simulink model "rfsoc4x2_ospfb_128"  (R2021a)
settings: Solver=VariableStepAuto  StartTime=0.0  StopTime=2048  RelTol=1e-3
undefined symbols (not defined in the file): pfb_coeff_gen_calc
libraries: xbsIndex_r4 x37092, casper_library_delays x737, casper_library_misc x68, xps_library x1
(part 83 of 339)

== system rfsoc4x2_ospfb_128/pfb_fir_real6/adder_1_12 ==
  sync : Inport
  din1 : Inport  Port=2
  din2 : Inport  Port=3
  din3 : Inport  Port=4
  din4 : Inport  Port=5
  addr1 : xbsIndex_r4/AddSub  mode=Addition  use_carryin=off  use_carryout=off  en=off  latency=1  precision=User Defined  arith_type="Signed  (2's comp)"  n_bits=32  bin_pt=30  quantization=Truncate  overflow=Wrap  use_behavioral_HDL=on  hw_selection=Fabric  pipelined=on  use_rpm=on  dbl_ovrd=off  block_type=addsub
  addr2 : xbsIndex_r4/AddSub  mode=Addition  use_carryin=off  use_carryout=off  en=off  latency=1  precision=User Defined  arith_type="Signed  (2's comp)"  n_bits=32  bin_pt=30  quantization=Truncate  overflow=Wrap  use_behavioral_HDL=on  hw_selection=Fabric  pipelined=on  use_rpm=on  dbl_ovrd=off  block_type=addsub
  addr3 : xbsIndex_r4/AddSub  mode=Addition  use_carryin=off  use_carryout=off  en=off  latency=1  precision=User Defined  arith_type="Signed  (2's comp)"  n_bits=32  bin_pt=30  quantization=Truncate  overflow=Wrap  use_behavioral_HDL=off  hw_selection=Fabric  pipelined=on  use_rpm=on  dbl_ovrd=off  block_type=addsub
  sync_delay : xbsIndex_r4/Delay  rst=off  infoeditControl=Selection of Reset will increase slice count due to use of real FFs and instead of SRLs  en=off  latency=2  reg_retiming=on  dbl_ovrd=off  block_type=delay
      settings: block_version=11.4
  sync_out : Outport  VectorParamsAs1DForOutWhenUnconnected=off
  dout : Outport  Port=2  VectorParamsAs1DForOutWhenUnconnected=off
  wires:
  sync/1 -> sync_delay/1
  sync_delay/1 -> sync_out/1
  din1/1 -> addr1/1
  din2/1 -> addr1/2
  din3/1 -> addr2/1
  din4/1 -> addr2/2
  addr1/1 -> addr3/1
  addr2/1 -> addr3/2
  addr3/1 -> dout/1

== system rfsoc4x2_ospfb_128/pfb_fir_real6/adder_1_13 ==
  sync : Inport
  din1 : Inport  Port=2
  din2 : Inport  Port=3
  din3 : Inport  Port=4
  din4 : Inport  Port=5
  addr1 : xbsIndex_r4/AddSub  mode=Addition  use_carryin=off  use_carryout=off  en=off  latency=1  precision=User Defined  arith_type="Signed  (2's comp)"  n_bits=32  bin_pt=30  quantization=Truncate  overflow=Wrap  use_behavioral_HDL=on  hw_selection=Fabric  pipelined=on  use_rpm=on  dbl_ovrd=off  block_type=addsub
  addr2 : xbsIndex_r4/AddSub  mode=Addition  use_carryin=off  use_carryout=off  en=off  latency=1  precision=User Defined  arith_type="Signed  (2's comp)"  n_bits=32  bin_pt=30  quantization=Truncate  overflow=Wrap  use_behavioral_HDL=on  hw_selection=Fabric  pipelined=on  use_rpm=on  dbl_ovrd=off  block_type=addsub
  addr3 : xbsIndex_r4/AddSub  mode=Addition  use_carryin=off  use_carryout=off  en=off  latency=1  precision=User Defined  arith_type="Signed  (2's comp)"  n_bits=32  bin_pt=30  quantization=Truncate  overflow=Wrap  use_behavioral_HDL=off  hw_selection=Fabric  pipelined=on  use_rpm=on  dbl_ovrd=off  block_type=addsub
  sync_delay : xbsIndex_r4/Delay  rst=off  infoeditControl=Selection of Reset will increase slice count due to use of real FFs and instead of SRLs  en=off  latency=2  reg_retiming=on  dbl_ovrd=off  block_type=delay
      settings: block_version=11.4
  sync_out : Outport  VectorParamsAs1DForOutWhenUnconnected=off
  dout : Outport  Port=2  VectorParamsAs1DForOutWhenUnconnected=off
  wires:
  sync/1 -> sync_delay/1
  sync_delay/1 -> sync_out/1
  din1/1 -> addr1/1
  din2/1 -> addr1/2
  din3/1 -> addr2/1
  din4/1 -> addr2/2
  addr1/1 -> addr3/1
  addr2/1 -> addr3/2
  addr3/1 -> dout/1

== system rfsoc4x2_ospfb_128/pfb_fir_real6/adder_1_14 ==
  sync : Inport
  din1 : Inport  Port=2
  din2 : Inport  Port=3
  din3 : Inport  Port=4
  din4 : Inport  Port=5
  addr1 : xbsIndex_r4/AddSub  mode=Addition  use_carryin=off  use_carryout=off  en=off  latency=1  precision=User Defined  arith_type="Signed  (2's comp)"  n_bits=32  bin_pt=30  quantization=Truncate  overflow=Wrap  use_behavioral_HDL=on  hw_selection=Fabric  pipelined=on  use_rpm=on  dbl_ovrd=off  block_type=addsub
  addr2 : xbsIndex_r4/AddSub  mode=Addition  use_carryin=off  use_carryout=off  en=off  latency=1  precision=User Defined  arith_type="Signed  (2's comp)"  n_bits=32  bin_pt=30  quantization=Truncate  overflow=Wrap  use_behavioral_HDL=on  hw_selection=Fabric  pipelined=on  use_rpm=on  dbl_ovrd=off  block_type=addsub
  addr3 : xbsIndex_r4/AddSub  mode=Addition  use_carryin=off  use_carryout=off  en=off  latency=1  precision=User Defined  arith_type="Signed  (2's comp)"  n_bits=32  bin_pt=30  quantization=Truncate  overflow=Wrap  use_behavioral_HDL=off  hw_selection=Fabric  pipelined=on  use_rpm=on  dbl_ovrd=off  block_type=addsub
  sync_delay : xbsIndex_r4/Delay  rst=off  infoeditControl=Selection of Reset will increase slice count due to use of real FFs and instead of SRLs  en=off  latency=2  reg_retiming=on  dbl_ovrd=off  block_type=delay
      settings: block_version=11.4
  sync_out : Outport  VectorParamsAs1DForOutWhenUnconnected=off
  dout : Outport  Port=2  VectorParamsAs1DForOutWhenUnconnected=off
  wires:
  sync/1 -> sync_delay/1
  sync_delay/1 -> sync_out/1
  din1/1 -> addr1/1
  din2/1 -> addr1/2
  din3/1 -> addr2/1
  din4/1 -> addr2/2
  addr1/1 -> addr3/1
  addr2/1 -> addr3/2
  addr3/1 -> dout/1

== system rfsoc4x2_ospfb_128/pfb_fir_real6/adder_1_15 ==
  sync : Inport
  din1 : Inport  Port=2
  din2 : Inport  Port=3
  din3 : Inport  Port=4
  din4 : Inport  Port=5
  addr1 : xbsIndex_r4/AddSub  mode=Addition  use_carryin=off  use_carryout=off  en=off  latency=1  precision=User Defined  arith_type="Signed  (2's comp)"  n_bits=32  bin_pt=30  quantization=Truncate  overflow=Wrap  use_behavioral_HDL=on  hw_selection=Fabric  pipelined=on  use_rpm=on  dbl_ovrd=off  block_type=addsub
  addr2 : xbsIndex_r4/AddSub  mode=Addition  use_carryin=off  use_carryout=off  en=off  latency=1  precision=User Defined  arith_type="Signed  (2's comp)"  n_bits=32  bin_pt=30  quantization=Truncate  overflow=Wrap  use_behavioral_HDL=on  hw_selection=Fabric  pipelined=on  use_rpm=on  dbl_ovrd=off  block_type=addsub
  addr3 : xbsIndex_r4/AddSub  mode=Addition  use_carryin=off  use_carryout=off  en=off  latency=1  precision=User Defined  arith_type="Signed  (2's comp)"  n_bits=32  bin_pt=30  quantization=Truncate  overflow=Wrap  use_behavioral_HDL=off  hw_selection=Fabric  pipelined=on  use_rpm=on  dbl_ovrd=off  block_type=addsub
  sync_delay : xbsIndex_r4/Delay  rst=off  infoeditControl=Selection of Reset will increase slice count due to use of real FFs and instead of SRLs  en=off  latency=2  reg_retiming=on  dbl_ovrd=off  block_type=delay
      settings: block_version=11.4
  sync_out : Outport  VectorParamsAs1DForOutWhenUnconnected=off
  dout : Outport  Port=2  VectorParamsAs1DForOutWhenUnconnected=off
  wires:
  sync/1 -> sync_delay/1
  sync_delay/1 -> sync_out/1
  din1/1 -> addr1/1
  din2/1 -> addr1/2
  din3/1 -> addr2/1
  din4/1 -> addr2/2
  addr1/1 -> addr3/1
  addr2/1 -> addr3/2
  addr3/1 -> dout/1

== system rfsoc4x2_ospfb_128/pfb_fir_real6/adder_1_16 ==
  sync : Inport
  din1 : Inport  Port=2
  din2 : Inport  Port=3
  din3 : Inport  Port=4
  din4 : Inport  Port=5
  addr1 : xbsIndex_r4/AddSub  mode=Addition  use_carryin=off  use_carryout=off  en=off  latency=1  precision=User Defined  arith_type="Signed  (2's comp)"  n_bits=32  bin_pt=30  quantization=Truncate  overflow=Wrap  use_behavioral_HDL=on  hw_selection=Fabric  pipelined=on  use_rpm=on  dbl_ovrd=off  block_type=addsub
  addr2 : xbsIndex_r4/AddSub  mode=Addition  use_carryin=off  use_carryout=off  en=off  latency=1  precision=User Defined  arith_type="Signed  (2's comp)"  n_bits=32  bin_pt=30  quantization=Truncate  overflow=Wrap  use_behavioral_HDL=on  hw_selection=Fabric  pipelined=on  use_rpm=on  dbl_ovrd=off  block_type=addsub
  addr3 : xbsIndex_r4/AddSub  mode=Addition  use_carryin=off  use_carryout=off  en=off  latency=1  precision=User Defined  arith_type="Signed  (2's comp)"  n_bits=32  bin_pt=30  quantization=Truncate  overflow=Wrap  use_behavioral_HDL=off  hw_selection=Fabric  pipelined=on  use_rpm=on  dbl_ovrd=off  block_type=addsub
  sync_delay : xbsIndex_r4/Delay  rst=off  infoeditControl=Selection of Reset will increase slice count due to use of real FFs and instead of SRLs  en=off  latency=2  reg_retiming=on  dbl_ovrd=off  block_type=delay
      settings: block_version=11.4
  sync_out : Outport  VectorParamsAs1DForOutWhenUnconnected=off
  dout : Outport  Port=2  VectorParamsAs1DForOutWhenUnconnected=off
  wires:
  sync/1 -> sync_delay/1
  sync_delay/1 -> sync_out/1
  din1/1 -> addr1/1
  din2/1 -> addr1/2
  din3/1 -> addr2/1
  din4/1 -> addr2/2
  addr1/1 -> addr3/1
  addr2/1 -> addr3/2
  addr3/1 -> dout/1

== system rfsoc4x2_ospfb_128/pfb_fir_real6/adder_1_2 ==
  sync : Inport
  din1 : Inport  Port=2
  din2 : Inport  Port=3
  din3 : Inport  Port=4
  din4 : Inport  Port=5
  addr1 : xbsIndex_r4/AddSub  mode=Addition  use_carryin=off  use_carryout=off  en=off  latency=1  precision=User Defined  arith_type="Signed  (2's comp)"  n_bits=32  bin_pt=30  quantization=Truncate  overflow=Wrap  use_behavioral_HDL=on  hw_selection=Fabric  pipelined=on  use_rpm=on  dbl_ovrd=off  block_type=addsub
  addr2 : xbsIndex_r4/AddSub  mode=Addition  use_carryin=off  use_carryout=off  en=off  latency=1  precision=User Defined  arith_type="Signed  (2's comp)"  n_bits=32  bin_pt=30  quantization=Truncate  overflow=Wrap  use_behavioral_HDL=on  hw_selection=Fabric  pipelined=on  use_rpm=on  dbl_ovrd=off  block_type=addsub
  addr3 : xbsIndex_r4/AddSub  mode=Addition  use_carryin=off  use_carryout=off  en=off  latency=1  precision=User Defined  arith_type="Signed  (2's comp)"  n_bits=32  bin_pt=30  quantization=Truncate  overflow=Wrap  use_behavioral_HDL=off  hw_selection=Fabric  pipelined=on  use_rpm=on  dbl_ovrd=off  block_type=addsub
  sync_delay : xbsIndex_r4/Delay  rst=off  infoeditControl=Selection of Reset will increase slice count due to use of real FFs and instead of SRLs  en=off  latency=2  reg_retiming=on  dbl_ovrd=off  block_type=delay
      settings: block_version=11.4
  sync_out : Outport  VectorParamsAs1DForOutWhenUnconnected=off
  dout : Outport  Port=2  VectorParamsAs1DForOutWhenUnconnected=off
  wires:
  sync/1 -> sync_delay/1
  sync_delay/1 -> sync_out/1
  din1/1 -> addr1/1
  din2/1 -> addr1/2
  din3/1 -> addr2/1
  din4/1 -> addr2/2
  addr1/1 -> addr3/1
  addr2/1 -> addr3/2
  addr3/1 -> dout/1

== system rfsoc4x2_ospfb_128/pfb_fir_real6/adder_1_3 ==
  sync : Inport
  din1 : Inport  Port=2
  din2 : Inport  Port=3
  din3 : Inport  Port=4
  din4 : Inport  Port=5
  addr1 : xbsIndex_r4/AddSub  mode=Addition  use_carryin=off  use_carryout=off  en=off  latency=1  precision=User Defined  arith_type="Signed  (2's comp)"  n_bits=32  bin_pt=30  quantization=Truncate  overflow=Wrap  use_behavioral_HDL=on  hw_selection=Fabric  pipelined=on  use_rpm=on  dbl_ovrd=off  block_type=addsub
  addr2 : xbsIndex_r4/AddSub  mode=Addition  use_carryin=off  use_carryout=off  en=off  latency=1  precision=User Defined  arith_type="Signed  (2's comp)"  n_bits=32  bin_pt=30  quantization=Truncate  overflow=Wrap  use_behavioral_HDL=on  hw_selection=Fabric  pipelined=on  use_rpm=on  dbl_ovrd=off  block_type=addsub
  addr3 : xbsIndex_r4/AddSub  mode=Addition  use_carryin=off  use_carryout=off  en=off  latency=1  precision=User Defined  arith_type="Signed  (2's comp)"  n_bits=32  bin_pt=30  quantization=Truncate  overflow=Wrap  use_behavioral_HDL=off  hw_selection=Fabric  pipelined=on  use_rpm=on  dbl_ovrd=off  block_type=addsub
  sync_delay : xbsIndex_r4/Delay  rst=off  infoeditControl=Selection of Reset will increase slice count due to use of real FFs and instead of SRLs  en=off  latency=2  reg_retiming=on  dbl_ovrd=off  block_type=delay
      settings: block_version=11.4
  sync_out : Outport  VectorParamsAs1DForOutWhenUnconnected=off
  dout : Outport  Port=2  VectorParamsAs1DForOutWhenUnconnected=off
  wires:
  sync/1 -> sync_delay/1
  sync_delay/1 -> sync_out/1
  din1/1 -> addr1/1
  din2/1 -> addr1/2
  din3/1 -> addr2/1
  din4/1 -> addr2/2
  addr1/1 -> addr3/1
  addr2/1 -> addr3/2
  addr3/1 -> dout/1

== system rfsoc4x2_ospfb_128/pfb_fir_real6/adder_1_4 ==
  sync : Inport
  din1 : Inport  Port=2
  din2 : Inport  Port=3
  din3 : Inport  Port=4
  din4 : Inport  Port=5
  addr1 : xbsIndex_r4/AddSub  mode=Addition  use_carryin=off  use_carryout=off  en=off  latency=1  precision=User Defined  arith_type="Signed  (2's comp)"  n_bits=32  bin_pt=30  quantization=Truncate  overflow=Wrap  use_behavioral_HDL=on  hw_selection=Fabric  pipelined=on  use_rpm=on  dbl_ovrd=off  block_type=addsub
  addr2 : xbsIndex_r4/AddSub  mode=Addition  use_carryin=off  use_carryout=off  en=off  latency=1  precision=User Defined  arith_type="Signed  (2's comp)"  n_bits=32  bin_pt=30  quantization=Truncate  overflow=Wrap  use_behavioral_HDL=on  hw_selection=Fabric  pipelined=on  use_rpm=on  dbl_ovrd=off  block_type=addsub
  addr3 : xbsIndex_r4/AddSub  mode=Addition  use_carryin=off  use_carryout=off  en=off  latency=1  precision=User Defined  arith_type="Signed  (2's comp)"  n_bits=32  bin_pt=30  quantization=Truncate  overflow=Wrap  use_behavioral_HDL=off  hw_selection=Fabric  pipelined=on  use_rpm=on  dbl_ovrd=off  block_type=addsub
  sync_delay : xbsIndex_r4/Delay  rst=off  infoeditControl=Selection of Reset will increase slice count due to use of real FFs and instead of SRLs  en=off  latency=2  reg_retiming=on  dbl_ovrd=off  block_type=delay
      settings: block_version=11.4
  sync_out : Outport  VectorParamsAs1DForOutWhenUnconnected=off
  dout : Outport  Port=2  VectorParamsAs1DForOutWhenUnconnected=off
  wires:
  sync/1 -> sync_delay/1
  sync_delay/1 -> sync_out/1
  din1/1 -> addr1/1
  din2/1 -> addr1/2
  din3/1 -> addr2/1
  din4/1 -> addr2/2
  addr1/1 -> addr3/1
  addr2/1 -> addr3/2
  addr3/1 -> dout/1

== system rfsoc4x2_ospfb_128/pfb_fir_real6/adder_1_5 ==
  sync : Inport
  din1 : Inport  Port=2
  din2 : Inport  Port=3
  din3 : Inport  Port=4
  din4 : Inport  Port=5
  addr1 : xbsIndex_r4/AddSub  mode=Addition  use_carryin=off  use_carryout=off  en=off  latency=1  precision=User Defined  arith_type="Signed  (2's comp)"  n_bits=32  bin_pt=30  quantization=Truncate  overflow=Wrap  use_behavioral_HDL=on  hw_selection=Fabric  pipelined=on  use_rpm=on  dbl_ovrd=off  block_type=addsub
  addr2 : xbsIndex_r4/AddSub  mode=Addition  use_carryin=off  use_carryout=off  en=off  latency=1  precision=User Defined  arith_type="Signed  (2's comp)"  n_bits=32  bin_pt=30  quantization=Truncate  overflow=Wrap  use_behavioral_HDL=on  hw_selection=Fabric  pipelined=on  use_rpm=on  dbl_ovrd=off  block_type=addsub
  addr3 : xbsIndex_r4/AddSub  mode=Addition  use_carryin=off  use_carryout=off  en=off  latency=1  precision=User Defined  arith_type="Signed  (2's comp)"  n_bits=32  bin_pt=30  quantization=Truncate  overflow=Wrap  use_behavioral_HDL=off  hw_selection=Fabric  pipelined=on  use_rpm=on  dbl_ovrd=off  block_type=addsub
  sync_delay : xbsIndex_r4/Delay  rst=off  infoeditControl=Selection of Reset will increase slice count due to use of real FFs and instead of SRLs  en=off  latency=2  reg_retiming=on  dbl_ovrd=off  block_type=delay
      settings: block_version=11.4
  sync_out : Outport  VectorParamsAs1DForOutWhenUnconnected=off
  dout : Outport  Port=2  VectorParamsAs1DForOutWhenUnconnected=off
  wires:
  sync/1 -> sync_delay/1
  sync_delay/1 -> sync_out/1
  din1/1 -> addr1/1
  din2/1 -> addr1/2
  din3/1 -> addr2/1
  din4/1 -> addr2/2
  addr1/1 -> addr3/1
  addr2/1 -> addr3/2
  addr3/1 -> dout/1

== system rfsoc4x2_ospfb_128/pfb_fir_real6/adder_1_6 ==
  sync : Inport
  din1 : Inport  Port=2
  din2 : Inport  Port=3
  din3 : Inport  Port=4
  din4 : Inport  Port=5
  addr1 : xbsIndex_r4/AddSub  mode=Addition  use_carryin=off  use_carryout=off  en=off  latency=1  precision=User Defined  arith_type="Signed  (2's comp)"  n_bits=32  bin_pt=30  quantization=Truncate  overflow=Wrap  use_behavioral_HDL=on  hw_selection=Fabric  pipelined=on  use_rpm=on  dbl_ovrd=off  block_type=addsub
  addr2 : xbsIndex_r4/AddSub  mode=Addition  use_carryin=off  use_carryout=off  en=off  latency=1  precision=User Defined  arith_type="Signed  (2's comp)"  n_bits=32  bin_pt=30  quantization=Truncate  overflow=Wrap  use_behavioral_HDL=on  hw_selection=Fabric  pipelined=on  use_rpm=on  dbl_ovrd=off  block_type=addsub
  addr3 : xbsIndex_r4/AddSub  mode=Addition  use_carryin=off  use_carryout=off  en=off  latency=1  precision=User Defined  arith_type="Signed  (2's comp)"  n_bits=32  bin_pt=30  quantization=Truncate  overflow=Wrap  use_behavioral_HDL=off  hw_selection=Fabric  pipelined=on  use_rpm=on  dbl_ovrd=off  block_type=addsub
  sync_delay : xbsIndex_r4/Delay  rst=off  infoeditControl=Selection of Reset will increase slice count due to use of real FFs and instead of SRLs  en=off  latency=2  reg_retiming=on  dbl_ovrd=off  block_type=delay
      settings: block_version=11.4
  sync_out : Outport  VectorParamsAs1DForOutWhenUnconnected=off
  dout : Outport  Port=2  VectorParamsAs1DForOutWhenUnconnected=off
  wires:
  sync/1 -> sync_delay/1
  sync_delay/1 -> sync_out/1
  din1/1 -> addr1/1
  din2/1 -> addr1/2
  din3/1 -> addr2/1
  din4/1 -> addr2/2
  addr1/1 -> addr3/1
  addr2/1 -> addr3/2
  addr3/1 -> dout/1

== system rfsoc4x2_ospfb_128/pfb_fir_real6/adder_1_7 ==
  sync : Inport
  din1 : Inport  Port=2
  din2 : Inport  Port=3
  din3 : Inport  Port=4
  din4 : Inport  Port=5
  addr1 : xbsIndex_r4/AddSub  mode=Addition  use_carryin=off  use_carryout=off  en=off  latency=1  precision=User Defined  arith_type="Signed  (2's comp)"  n_bits=32  bin_pt=30  quantization=Truncate  overflow=Wrap  use_behavioral_HDL=on  hw_selection=Fabric  pipelined=on  use_rpm=on  dbl_ovrd=off  block_type=addsub
  addr2 : xbsIndex_r4/AddSub  mode=Addition  use_carryin=off  use_carryout=off  en=off  latency=1  precision=User Defined  arith_type="Signed  (2's comp)"  n_bits=32  bin_pt=30  quantization=Truncate  overflow=Wrap  use_behavioral_HDL=on  hw_selection=Fabric  pipelined=on  use_rpm=on  dbl_ovrd=off  block_type=addsub
  addr3 : xbsIndex_r4/AddSub  mode=Addition  use_carryin=off  use_carryout=off  en=off  latency=1  precision=User Defined  arith_type="Signed  (2's comp)"  n_bits=32  bin_pt=30  quantization=Truncate  overflow=Wrap  use_behavioral_HDL=off  hw_selection=Fabric  pipelined=on  use_rpm=on  dbl_ovrd=off  block_type=addsub
  sync_delay : xbsIndex_r4/Delay  rst=off  infoeditControl=Selection of Reset will increase slice count due to use of real FFs and instead of SRLs  en=off  latency=2  reg_retiming=on  dbl_ovrd=off  block_type=delay
      settings: block_version=11.4
  sync_out : Outport  VectorParamsAs1DForOutWhenUnconnected=off
  dout : Outport  Port=2  VectorParamsAs1DForOutWhenUnconnected=off
  wires:
  sync/1 -> sync_delay/1
  sync_delay/1 -> sync_out/1
  din1/1 -> addr1/1
  din2/1 -> addr1/2
  din3/1 -> addr2/1
  din4/1 -> addr2/2
  addr1/1 -> addr3/1
  addr2/1 -> addr3/2
  addr3/1 -> dout/1

== system rfsoc4x2_ospfb_128/pfb_fir_real6/adder_1_8 ==
  sync : Inport
  din1 : Inport  Port=2
  din2 : Inport  Port=3
  din3 : Inport  Port=4
  din4 : Inport  Port=5
  addr1 : xbsIndex_r4/AddSub  mode=Addition  use_carryin=off  use_carryout=off  en=off  latency=1  precision=User Defined  arith_type="Signed  (2's comp)"  n_bits=32  bin_pt=30  quantization=Truncate  overflow=Wrap  use_behavioral_HDL=on  hw_selection=Fabric  pipelined=on  use_rpm=on  dbl_ovrd=off  block_type=addsub
  addr2 : xbsIndex_r4/AddSub  mode=Addition  use_carryin=off  use_carryout=off  en=off  latency=1  precision=User Defined  arith_type="Signed  (2's comp)"  n_bits=32  bin_pt=30  quantization=Truncate  overflow=Wrap  use_behavioral_HDL=on  hw_selection=Fabric  pipelined=on  use_rpm=on  dbl_ovrd=off  block_type=addsub
  addr3 : xbsIndex_r4/AddSub  mode=Addition  use_carryin=off  use_carryout=off  en=off  latency=1  precision=User Defined  arith_type="Signed  (2's comp)"  n_bits=32  bin_pt=30  quantization=Truncate  overflow=Wrap  use_behavioral_HDL=off  hw_selection=Fabric  pipelined=on  use_rpm=on  dbl_ovrd=off  block_type=addsub
  sync_delay : xbsIndex_r4/Delay  rst=off  infoeditControl=Selection of Reset will increase slice count due to use of real FFs and instead of SRLs  en=off  latency=2  reg_retiming=on  dbl_ovrd=off  block_type=delay
      settings: block_version=11.4
  sync_out : Outport  VectorParamsAs1DForOutWhenUnconnected=off
  dout : Outport  Port=2  VectorParamsAs1DForOutWhenUnconnected=off
  wires:
  sync/1 -> sync_delay/1
  sync_delay/1 -> sync_out/1
  din1/1 -> addr1/1
  din2/1 -> addr1/2
  din3/1 -> addr2/1
  din4/1 -> addr2/2
  addr1/1 -> addr3/1
  addr2/1 -> addr3/2
  addr3/1 -> dout/1

== system rfsoc4x2_ospfb_128/pfb_fir_real6/adder_1_9 ==
  sync : Inport
  din1 : Inport  Port=2
  din2 : Inport  Port=3
  din3 : Inport  Port=4
  din4 : Inport  Port=5
  addr1 : xbsIndex_r4/AddSub  mode=Addition  use_carryin=off  use_carryout=off  en=off  latency=1  precision=User Defined  arith_type="Signed  (2's comp)"  n_bits=32  bin_pt=30  quantization=Truncate  overflow=Wrap  use_behavioral_HDL=on  hw_selection=Fabric  pipelined=on  use_rpm=on  dbl_ovrd=off  block_type=addsub
  addr2 : xbsIndex_r4/AddSub  mode=Addition  use_carryin=off  use_carryout=off  en=off  latency=1  precision=User Defined  arith_type="Signed  (2's comp)"  n_bits=32  bin_pt=30  quantization=Truncate  overflow=Wrap  use_behavioral_HDL=on  hw_selection=Fabric  pipelined=on  use_rpm=on  dbl_ovrd=off  block_type=addsub
  addr3 : xbsIndex_r4/AddSub  mode=Addition  use_carryin=off  use_carryout=off  en=off  latency=1  precision=User Defined  arith_type="Signed  (2's comp)"  n_bits=32  bin_pt=30  quantization=Truncate  overflow=Wrap  use_behavioral_HDL=off  hw_selection=Fabric  pipelined=on  use_rpm=on  dbl_ovrd=off  block_type=addsub
  sync_delay : xbsIndex_r4/Delay  rst=off  infoeditControl=Selection of Reset will increase slice count due to use of real FFs and instead of SRLs  en=off  latency=2  reg_retiming=on  dbl_ovrd=off  block_type=delay
      settings: block_version=11.4
  sync_out : Outport  VectorParamsAs1DForOutWhenUnconnected=off
  dout : Outport  Port=2  VectorParamsAs1DForOutWhenUnconnected=off
  wires:
  sync/1 -> sync_delay/1
  sync_delay/1 -> sync_out/1
  din1/1 -> addr1/1
  din2/1 -> addr1/2
  din3/1 -> addr2/1
  din4/1 -> addr2/2
  addr1/1 -> addr3/1
  addr2/1 -> addr3/2
  addr3/1 -> dout/1

== system rfsoc4x2_ospfb_128/pfb_fir_real6/edge_detect8 ==
  in : Inport
  Delay : xbsIndex_r4/Delay  rst=off  infoeditControl=Selection of Reset will increase slice count due to use of real FFs and instead of SRLs  en=off  latency=1  reg_retiming=off  dbl_ovrd=off  block_type=delay
      settings: xl_area=[0, 0, 0, 0, 0, 0, 0]
  Inverter : xbsIndex_r4/Inverter  en=off  latency=0  dbl_ovrd=off  block_type=inv
      settings: xl_area=[0, 0, 0, 0, 0, 0, 0]
  edge_op : xbsIndex_r4/Logical  logical_function=AND  inputs=2  en=off  latency=0  precision=Full  arith_type=Unsigned  n_bits=8  bin_pt=2  align_bp=on  dbl_ovrd=off  block_type=logical
      settings: xl_area=[0, 0, 0, 0, 0, 0, 0]
  out : Outport  VectorParamsAs1DForOutWhenUnconnected=off
  wires:
  Inverter/1 -> edge_op/1
  edge_op/1 -> out/1
  in/1 -> Inverter/1, Delay/1
  Delay/1 -> edge_op/2

== system rfsoc4x2_ospfb_128/pfb_fir_real6/pol1_in1_coeffs ==
  din : Inport
  sync : Inport  Port=2
  Concat : xbsIndex_r4/Concat  num_inputs=4  dbl_ovrd=off  block_type=concat
      settings: block_version=9.1.01
  Counter : xbsIndex_r4/Counter  cnt_type=Free Running  cnt_to=Inf  operation=Up  start_count=0  cnt_by_val=1  arith_type=Unsigned  n_bits=4  bin_pt=0  load_pin=off  rst=on  en=off  explicit_period=on  period=1  use_behavioral_HDL=off  implementation=Fabric  use_rpm=on  dbl_ovrd=off  block_type=counter
      settings: xl_area=[0, 0, 0, 0, 0, 0, 0]  block_version=9.1.01
  Delay : xbsIndex_r4/Delay  rst=off  infoeditControl=Selection of Reset will increase slice count due to use of real FFs and instead of SRLs  en=off  latency=bram_latency+1+fan_latency  reg_retiming=off  dbl_ovrd=off  block_type=delay
      settings: xl_area=[0, 0, 0, 0, 0, 0, 0]  block_version=9.1.01
  Delay1 : xbsIndex_r4/Delay  rst=off  infoeditControl=Selection of Reset will increase slice count due to use of real FFs and instead of SRLs  en=off  latency=bram_latency+1+fan_latency  reg_retiming=off  dbl_ovrd=off  block_type=delay
      settings: xl_area=[0, 0, 0, 0, 0, 0, 0]  block_version=9.1.01
  ROM1 : xbsIndex_r4/ROM  depth=16  initVector=pfb_coeff_gen_calc(8, 4,'hamming',4, 0,1.1599999999999999200639422269887,1,false)  distributed_mem=Block RAM  rst=off  init_reg=0  en=off  latency=bram_latency  gui_display_data_type=Fixed-point  arith_type="Signed  (2's comp)"  n_bits=16  bin_pt=15  preci_type=Single  exp_width=8  frac_width=24  optimize=Area  use_rpm=on  dbl_ovrd=off  simulation_type=fast_sim  block_type=sprom
      settings: xl_area=[0, 0, 0, 0, 0, 0, 0]
  ROM2 : xbsIndex_r4/ROM  depth=16  initVector=pfb_coeff_gen_calc(8, 4,'hamming',4, 0,1.1599999999999999200639422269887,2,false)  distributed_mem=Block RAM  rst=off  init_reg=0  en=off  latency=bram_latency  gui_display_data_type=Fixed-point  arith_type="Signed  (2's comp)"  n_bits=16  bin_pt=15  preci_type=Single  exp_width=8  frac_width=24  optimize=Area  use_rpm=on  dbl_ovrd=off  simulation_type=fast_sim  block_type=sprom
      settings: xl_area=[0, 0, 0, 0, 0, 0, 0]
  ROM3 : xbsIndex_r4/ROM  depth=16  initVector=pfb_coeff_gen_calc(8, 4,'hamming',4, 0,1.1599999999999999200639422269887,3,false)  distributed_mem=Block RAM  rst=off  init_reg=0  en=off  latency=bram_latency  gui_display_data_type=Fixed-point  arith_type="Signed  (2's comp)"  n_bits=16  bin_pt=15  preci_type=Single  exp_width=8  frac_width=24  optimize=Area  use_rpm=on  dbl_ovrd=off  simulation_type=fast_sim  block_type=sprom
  ROM4 : xbsIndex_r4/ROM  depth=16  initVector=pfb_coeff_gen_calc(8, 4,'hamming',4, 0,1.1599999999999999200639422269887,4,false)  distributed_mem=Block RAM  rst=off  init_reg=0  en=off  latency=bram_latency  gui_display_data_type=Fixed-point  arith_type="Signed  (2's comp)"  n_bits=16  bin_pt=15  preci_type=Single  exp_width=8  frac_width=24  optimize=Area  use_rpm=on  dbl_ovrd=off  simulation_type=fast_sim  block_type=sprom
  Register : xbsIndex_r4/Register  init=0  rst=off  en=off  dbl_ovrd=off  block_type=register
      settings: xl_area=[0, 0, 0, 0, 0, 0, 0]  block_version=9.1.01
  Reinterpret{1..4} (4 alike) : xbsIndex_r4/Reinterpret  force_arith_type=on  arith_type=Unsigned  force_bin_pt=on  bin_pt=0  block_type=reinterpret
      Reinterpret1 settings: infoedit="Changes signal type without altering the binary representation.   You can changed the signal between signed and unsigned, and relocate the binary point.<P><P>Hardware notes: In hardware this block costs nothing.<P><P>Example:  Suppose the input is 6 bits wide, signed, with 2 fractional bits, and the output is forced to unsigned with 0 fractional bits.  Then an input of -2.0 (1110.00 in binary 2's complement) becomes an output of 56 (111000 in binary)."  block_version=9.1.01
      Reinterpret2 settings: infoedit="Changes signal type without altering the binary representation.   You can changed the signal between signed and unsigned, and relocate the binary point.<P><P>Hardware notes: In hardware this block costs nothing.<P><P>Example:  Suppose the input is 6 bits wide, signed, with 2 fractional bits, and the output is forced to unsigned with 0 fractional bits.  Then an input of -2.0 (1110.00 in binary 2's complement) becomes an output of 56 (111000 in binary)."  block_version=9.1.01
  fan_delay{1..4} (4 alike) : xbsIndex_r4/Delay  rst=off  infoeditControl=Selection of Reset will increase slice count due to use of real FFs and instead of SRLs  en=off  latency=fan_latency  reg_retiming=off  dbl_ovrd=off  block_type=delay
      fan_delay1 settings: block_version=11.4
      fan_delay2 settings: block_version=11.4
  dout : Outport  VectorParamsAs1DForOutWhenUnconnected=off
  sync_out : Outport  Port=2  VectorParamsAs1DForOutWhenUnconnected=off
  coeff : Outport  Port=3  VectorParamsAs1DForOutWhenUnconnected=off
  wires:
  din/1 -> Delay1/1
  Delay1/1 -> dout/1
  sync/1 -> Counter/1, Delay/1
  Delay/1 -> sync_out/1
  Concat/1 -> Register/1
  Register/1 -> coeff/1
  Counter/1 -> fan_delay1/1, fan_delay2/1, fan_delay3/1, fan_delay4/1
  fan_delay1/1 -> ROM1/1
  ROM1/1 -> Reinterpret1/1
  Reinterpret1/1 -> Concat/1
  fan_delay2/1 -> ROM2/1
  ROM2/1 -> Reinterpret2/1
  Reinterpret2/1 -> Concat/2
  fan_delay3/1 -> ROM3/1
  ROM3/1 -> Reinterpret3/1
  Reinterpret3/1 -> Concat/3
  fan_delay4/1 -> ROM4/1
  ROM4/1 -> Reinterpret4/1
  Reinterpret4/1 -> Concat/4

== system rfsoc4x2_ospfb_128/pfb_fir_real6/pol1_in1_first_tap ==
  note: 10 data out
  note: 9 data in
  note: 9 data out
  din : Inport
  sync : Inport  Port=2
  coeffs : Inport  Port=3
  addr_in : Inport  Port=4
  pot_en_in : Inport  Port=5
  Constant59 : xbsIndex_r4/Constant  const=0  gui_display_data_type=Fixed-point  arith_type=Unsigned  n_bits=16  bin_pt=0  preci_type=Single  exp_width=8  frac_width=24  explicit_period=off  period=1  equ=P=C  opselect=C  inp2=PCIN>>17  opr=+  inp1=P  carry=CIN  dbl_ovrd=off  block_type=constant
  Constant60 : xbsIndex_r4/Constant  const=0  gui_display_data_type=Boolean  arith_type=Boolean  n_bits=144  bin_pt=0  preci_type=Single  exp_width=8  frac_width=24  explicit_period=off  period=1  equ=P=C  opselect=C  inp2=PCIN>>17  opr=+  inp1=P  carry=CIN  dbl_ovrd=off  block_type=constant
  Delay : xbsIndex_r4/Delay  rst=off  infoeditControl=Selection of Reset will increase slice count due to use of real FFs and instead of SRLs  en=off  latency=1  reg_retiming=off  dbl_ovrd=off  block_type=delay
  Delay1 : xbsIndex_r4/Delay  rst=off  infoeditControl=Selection of Reset will increase slice count due to use of real FFs and instead of SRLs  en=off  latency=1  reg_retiming=off  dbl_ovrd=off  block_type=delay
  Delay2 : xbsIndex_r4/Delay  rst=off  infoeditControl=Selection of Reset will increase slice count due to use of real FFs and instead of SRLs  en=off  latency=1  reg_retiming=off  dbl_ovrd=off  block_type=delay
  Dual Port RAM13 : xbsIndex_r4/Dual Port RAM  depth=(2^8) / (2^4)  initVector=0  distributed_mem=Block RAM  init_a=0  init_b=0  rst_a=off  rst_b=off  en_a=off  en_b=off  latency=1  write_mode_A=Read After Write  write_mode_B=Read Before Write  optimize=Area  dbl_ovrd=off  simulation_type=fast_sim  block_type=dpram
  Gateway Out1 : xbsIndex_r4/Gateway Out  inherit_from_input=off  hdl_port=on  rows=1  columns=1  UseAsDAC=off  DACChannel='1'  interface=None  automatic_assignment=on  address_offset=hex2dec('00')  intf_name=''  intf_description=''  timing_constraint=None  locs_specified=off  LOCs={}  io_standard={}  block_type=gatewayout
  Gateway Out3 : xbsIndex_r4/Gateway Out  inherit_from_input=off  hdl_port=on  rows=1  columns=1  UseAsDAC=off  DACChannel='1'  interface=None  automatic_assignment=on  address_offset=hex2dec('00')  intf_name=''  intf_description=''  timing_constraint=None  locs_specified=off  LOCs={}  io_standard={}  block_type=gatewayout
  Gateway Out4 : xbsIndex_r4/Gateway Out  inherit_from_input=off  hdl_port=on  rows=1  columns=1  UseAsDAC=off  DACChannel='1'  interface=None  automatic_assignment=on  address_offset=hex2dec('00')  intf_name=''  intf_description=''  timing_constraint=None  locs_specified=off  LOCs={}  io_standard={}  block_type=gatewayout
  Mult : xbsIndex_r4/Mult  precision=Full  arith_type="Signed  (2's comp)"  n_bits=8  bin_pt=2  quantization=Truncate  overflow=Wrap  en=off  latency=0  use_behavioral_HDL=on  opt=Speed  use_embedded=off  optimum_pipeline=off  pipeline=on  dbl_ovrd=off  use_rpm=on  placement_style=Rectangular shape  block_type=mult
      settings: xl_area=[0, 0, 0, 0, 0, 0, 0]  block_version=9.1.01
  Mult1 : xbsIndex_r4/Mult  Commented=on  precision=Full  arith_type="Signed  (2's comp)"  n_bits=8  bin_pt=2  quantization=Truncate  overflow=Wrap  en=off  latency=mult_latency  use_behavioral_HDL=on  opt=Speed  use_embedded=off  optimum_pipeline=off  pipeline=on  dbl_ovrd=off  use_rpm=on  placement_style=Rectangular shape  block_type=mult
      settings: infoedit=Hardware notes: To use the internal pipeline stage of the dedicated multiplier you must select 'Pipeline for maximum performance'.  xl_area=[0, 0, 0, 0, 0, 0, 0]  block_version=9.1.01
  Reinterpret : xbsIndex_r4/Reinterpret  force_arith_type=on  arith_type="Signed  (2's comp)"  force_bin_pt=on  bin_pt=CoeffBitWidth - 1  block_type=reinterpret
      settings: infoedit="Changes signal type without altering the binary representation.   You can changed the signal between signed and unsigned, and relocate the binary point.<P><P>Hardware notes: In hardware this block costs nothing.<P><P>Example:  Suppose the input is 6 bits wide, signed, with 2 fractional bits, and the output is forced to unsigned with 0 fractional bits.  Then an input of -2.0 (1110.00 in binary 2's complement) becomes an output of 56 (111000 in binary)."  block_version=9.1.01
  Reinterpret2 : xbsIndex_r4/Reinterpret  force_arith_type=on  arith_type="Signed  (2's comp)"  force_bin_pt=on  bin_pt=BitWidthIn - 1  block_type=reinterpret
      settings: infoedit="Changes signal type without altering the binary representation.   You can changed the signal between signed and unsigned, and relocate the binary point.<P><P>Hardware notes: In hardware this block costs nothing.<P><P>Example:  Suppose the input is 6 bits wide, signed, with 2 fractional bits, and the output is forced to unsigned with 0 fractional bits.  Then an input of -2.0 (1110.00 in binary 2's complement) becomes an output of 56 (111000 in binary)."  block_version=9.1.01
  Slice : xbsIndex_r4/Slice  nbits=CoeffBitWidth  boolean_output=off  mode=Lower Bit Location + Width  bit1=0  base1=MSB of Input  bit0=0  base0=LSB of Input  dbl_ovrd=off  block_type=slice
      settings: infoedit="Extracts a given range of bits from each input sample and presents it at the output.  The output type is ordinarily unsigned with binary point at zero, but can be Boolean when the slice is one bit wide.<P><P>Hardware notes: In hardware this block costs nothing."  block_version=9.1.01
  Slice1 : xbsIndex_r4/Slice  nbits=CoeffBitWidth * (TotalTaps - 1)  boolean_output=off  mode=Two Bit Locations  bit1=0  base1=MSB of Input  bit0=CoeffBitWidth  base0=LSB of Input  dbl_ovrd=off  block_type=slice
      settings: infoedit="Extracts a given range of bits from each input sample and presents it at the output.  The output type is ordinarily unsigned with binary point at zero, but can be Boolean when the slice is one bit wide.<P><P>Hardware notes: In hardware this block costs nothing."  block_version=9.1.01
  Terminator13 : Terminator
  scope1 : Scope
  scope2 : Scope  NumInputPorts=2
  sync_delay : casper_library_delays/sync_delay  DelayLen=2^(PFBSize-n_inputs) * n_pol_blocks
      settings: SourceProductName=CASPER DSP Blockset
  dout : Outport  VectorParamsAs1DForOutWhenUnconnected=off
  sync_out : Outport  Port=2  VectorParamsAs1DForOutWhenUnconnected=off
  coeff_out : Outport  Port=3  VectorParamsAs1DForOutWhenUnconnected=off
  taps_out : Outport  Port=4  VectorParamsAs1DForOutWhenUnconnected=off
  add_out : Outport  Port=5  VectorParamsAs1DForOutWhenUnconnected=off
  pot_en_out : Outport  Port=6  VectorParamsAs1DForOutWhenUnconnected=off
  wires:
  coeffs/1 -> Slice1/1, Slice/1
  Reinterpret2/1 -> Mult/1
  Reinterpret/1 -> Gateway Out3/1, Mult/2
  Slice/1 -> Reinterpret/1
  Slice1/1 -> Delay2/1
  sync_delay/1 -> sync_out/1
  Dual Port RAM13/2 -> dout/1
  Mult/1 -> taps_out/1
  sync/1 -> sync_delay/1
  din/1 -> Dual Port RAM13/2, Reinterpret2/1, Gateway Out4/1
  pot_en_in/1 -> Delay1/1, Dual Port RAM13/3
  Constant59/1 -> Dual Port RAM13/5
  Constant60/1 -> Dual Port RAM13/6
  addr_in/1 -> Delay/1, Dual Port RAM13/4, Gateway Out1/1, Dual Port RAM13/1
  Dual Port RAM13/1 -> Terminator13/1
  Delay/1 -> add_out/1
  Delay1/1 -> pot_en_out/1
  Gateway Out1/1 -> scope1/1
  Gateway Out3/1 -> scope2/2
  Gateway Out4/1 -> scope2/1
  Delay2/1 -> coeff_out/1

== system rfsoc4x2_ospfb_128/pfb_fir_real6/pol1_in1_first_tap1 ==
  note: 10 data out
  note: 9 data in
  note: 9 data out
  din : Inport
  sync : Inport  Port=2
  coeffs : Inport  Port=3
  addr_in : Inport  Port=4
  pot_en_in : Inport  Port=5
  Constant59 : xbsIndex_r4/Constant  const=0  gui_display_data_type=Fixed-point  arith_type=Unsigned  n_bits=16  bin_pt=0  preci_type=Single  exp_width=8  frac_width=24  explicit_period=off  period=1  equ=P=C  opselect=C  inp2=PCIN>>17  opr=+  inp1=P  carry=CIN  dbl_ovrd=off  block_type=constant
  Constant60 : xbsIndex_r4/Constant  const=0  gui_display_data_type=Boolean  arith_type=Boolean  n_bits=144  bin_pt=0  preci_type=Single  exp_width=8  frac_width=24  explicit_period=off  period=1  equ=P=C  opselect=C  inp2=PCIN>>17  opr=+  inp1=P  carry=CIN  dbl_ovrd=off  block_type=constant
  Delay : xbsIndex_r4/Delay  rst=off  infoeditControl=Selection of Reset will increase slice count due to use of real FFs and instead of SRLs  en=off  latency=1  reg_retiming=off  dbl_ovrd=off  block_type=delay
  Delay1 : xbsIndex_r4/Delay  rst=off  infoeditControl=Selection of Reset will increase slice count due to use of real FFs and instead of SRLs  en=off  latency=1  reg_retiming=off  dbl_ovrd=off  block_type=delay
  Delay2 : xbsIndex_r4/Delay  rst=off  infoeditControl=Selection of Reset will increase slice count due to use of real FFs and instead of SRLs  en=off  latency=1  reg_retiming=off  dbl_ovrd=off  block_type=delay
  Dual Port RAM13 : xbsIndex_r4/Dual Port RAM  depth=(2^8) / (2^4)  initVector=0  distributed_mem=Block RAM  init_a=0  init_b=0  rst_a=off  rst_b=off  en_a=off  en_b=off  latency=1  write_mode_A=Read After Write  write_mode_B=Read Before Write  optimize=Area  dbl_ovrd=off  simulation_type=fast_sim  block_type=dpram
  Gateway Out1 : xbsIndex_r4/Gateway Out  inherit_from_input=off  hdl_port=on  rows=1  columns=1  UseAsDAC=off  DACChannel='1'  interface=None  automatic_assignment=on  address_offset=hex2dec('00')  intf_name=''  intf_description=''  timing_constraint=None  locs_specified=off  LOCs={}  io_standard={}  block_type=gatewayout
  Gateway Out3 : xbsIndex_r4/Gateway Out  inherit_from_input=off  hdl_port=on  rows=1  columns=1  UseAsDAC=off  DACChannel='1'  interface=None  automatic_assignment=on  address_offset=hex2dec('00')  intf_name=''  intf_description=''  timing_constraint=None  locs_specified=off  LOCs={}  io_standard={}  block_type=gatewayout
  Gateway Out4 : xbsIndex_r4/Gateway Out  inherit_from_input=off  hdl_port=on  rows=1  columns=1  UseAsDAC=off  DACChannel='1'  interface=None  automatic_assignment=on  address_offset=hex2dec('00')  intf_name=''  intf_description=''  timing_constraint=None  locs_specified=off  LOCs={}  io_standard={}  block_type=gatewayout
  Mult : xbsIndex_r4/Mult  precision=Full  arith_type="Signed  (2's comp)"  n_bits=8  bin_pt=2  quantization=Truncate  overflow=Wrap  en=off  latency=0  use_behavioral_HDL=on  opt=Speed  use_embedded=off  optimum_pipeline=off  pipeline=on  dbl_ovrd=off  use_rpm=on  placement_style=Rectangular shape  block_type=mult
      settings: xl_area=[0, 0, 0, 0, 0, 0, 0]  block_version=9.1.01
  Mult1 : xbsIndex_r4/Mult  Commented=on  precision=Full  arith_type="Signed  (2's comp)"  n_bits=8  bin_pt=2  quantization=Truncate  overflow=Wrap  en=off  latency=mult_latency  use_behavioral_HDL=on  opt=Speed  use_embedded=off  optimum_pipeline=off  pipeline=on  dbl_ovrd=off  use_rpm=on  placement_style=Rectangular shape  block_type=mult
      settings: infoedit=Hardware notes: To use the internal pipeline stage of the dedicated multiplier you must select 'Pipeline for maximum performance'.  xl_area=[0, 0, 0, 0, 0, 0, 0]  block_version=9.1.01
  Reinterpret : xbsIndex_r4/Reinterpret  force_arith_type=on  arith_type="Signed  (2's comp)"  force_bin_pt=on  bin_pt=CoeffBitWidth - 1  block_type=reinterpret
      settings: infoedit="Changes signal type without altering the binary representation.   You can changed the signal between signed and unsigned, and relocate the binary point.<P><P>Hardware notes: In hardware this block costs nothing.<P><P>Example:  Suppose the input is 6 bits wide, signed, with 2 fractional bits, and the output is forced to unsigned with 0 fractional bits.  Then an input of -2.0 (1110.00 in binary 2's complement) becomes an output of 56 (111000 in binary)."  block_version=9.1.01
  Reinterpret2 : xbsIndex_r4/Reinterpret  force_arith_type=on  arith_type="Signed  (2's comp)"  force_bin_pt=on  bin_pt=BitWidthIn - 1  block_type=reinterpret
      settings: infoedit="Changes signal type without altering the binary representation.   You can changed the signal between signed and unsigned, and relocate the binary point.<P><P>Hardware notes: In hardware this block costs nothing.<P><P>Example:  Suppose the input is 6 bits wide, signed, with 2 fractional bits, and the output is forced to unsigned with 0 fractional bits.  Then an input of -2.0 (1110.00 in binary 2's complement) becomes an output of 56 (111000 in binary)."  block_version=9.1.01
  Slice : xbsIndex_r4/Slice  nbits=CoeffBitWidth  boolean_output=off  mode=Lower Bit Location + Width  bit1=0  base1=MSB of Input  bit0=0  base0=LSB of Input  dbl_ovrd=off  block_type=slice
      settings: infoedit="Extracts a given range of bits from each input sample and presents it at the output.  The output type is ordinarily unsigned with binary point at zero, but can be Boolean when the slice is one bit wide.<P><P>Hardware notes: In hardware this block costs nothing."  block_version=9.1.01
  Slice1 : xbsIndex_r4/Slice  nbits=CoeffBitWidth * (TotalTaps - 1)  boolean_output=off  mode=Two Bit Locations  bit1=0  base1=MSB of Input  bit0=CoeffBitWidth  base0=LSB of Input  dbl_ovrd=off  block_type=slice
      settings: infoedit="Extracts a given range of bits from each input sample and presents it at the output.  The output type is ordinarily unsigned with binary point at zero, but can be Boolean when the slice is one bit wide.<P><P>Hardware notes: In hardware this block costs nothing."  block_version=9.1.01
  Terminator13 : Terminator
  scope1 : Scope
  scope2 : Scope  NumInputPorts=2
  sync_delay : casper_library_delays/sync_delay  DelayLen=2^(PFBSize-n_inputs) * n_pol_blocks
      settings: SourceProductName=CASPER DSP Blockset
  dout : Outport  VectorParamsAs1DForOutWhenUnconnected=off
  sync_out : Outport  Port=2  VectorParamsAs1DForOutWhenUnconnected=off
  coeff_out : Outport  Port=3  VectorParamsAs1DForOutWhenUnconnected=off
  taps_out : Outport  Port=4  VectorParamsAs1DForOutWhenUnconnected=off
  add_out : Outport  Port=5  VectorParamsAs1DForOutWhenUnconnected=off
  pot_en_out : Outport  Port=6  VectorParamsAs1DForOutWhenUnconnected=off
  wires:
  coeffs/1 -> Slice1/1, Slice/1
  Reinterpret2/1 -> Mult/1
  Reinterpret/1 -> Gateway Out3/1, Mult/2
  Slice/1 -> Reinterpret/1
  Slice1/1 -> Delay2/1
  sync_delay/1 -> sync_out/1
  Dual Port RAM13/2 -> dout/1
  Mult/1 -> taps_out/1
  sync/1 -> sync_delay/1
  din/1 -> Dual Port RAM13/2, Reinterpret2/1, Gateway Out4/1
  pot_en_in/1 -> Delay1/1, Dual Port RAM13/3
  Constant59/1 -> Dual Port RAM13/5
  Constant60/1 -> Dual Port RAM13/6
  addr_in/1 -> Delay/1, Dual Port RAM13/4, Gateway Out1/1, Dual Port RAM13/1
  Dual Port RAM13/1 -> Terminator13/1
  Delay/1 -> add_out/1
  Delay1/1 -> pot_en_out/1
  Gateway Out1/1 -> scope1/1
  Gateway Out3/1 -> scope2/2
  Gateway Out4/1 -> scope2/1
  Delay2/1 -> coeff_out/1
